simulink model "furuta_observer_loop"  (R2024b)
settings: Solver=ode45  StartTime=0.0  StopTime=4  MaxStep=1e-3  RelTol=1e-3
values from neighbouring files (symbols this model uses):
  L = place(A', C', p_obs)'    [furuta_observer.m]
  tap_amp = 1    [furuta_no_observer.m]    (also in furuta_observer.m)
  tap_len = 0.1    [furuta_no_observer.m]    (also in furuta_observer.m)
  tap_time = 2    [furuta_no_observer.m]    (also in furuta_observer.m)
  Vmax = 10    [furuta_no_observer.m]    (also in furuta_observer.m)
  x0 = [0; deg2rad(10); 0; 0]    [furuta_no_observer.m]    (also in furuta_observer.m)
  xhat0 = zeros(4,1)    [furuta_observer.m]
undefined symbols (not defined in the file or in its folder): A, B, C, K
settings Model: Creator=alekseiprakhiy  LastModifiedBy=alekseiprakhiy

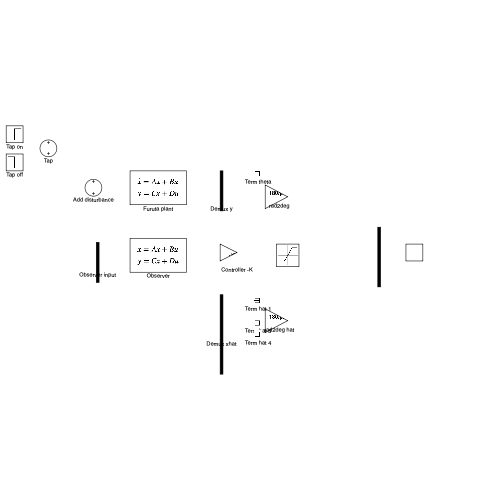
[thumbnail: Simulink's stored preview of the top-level diagram]
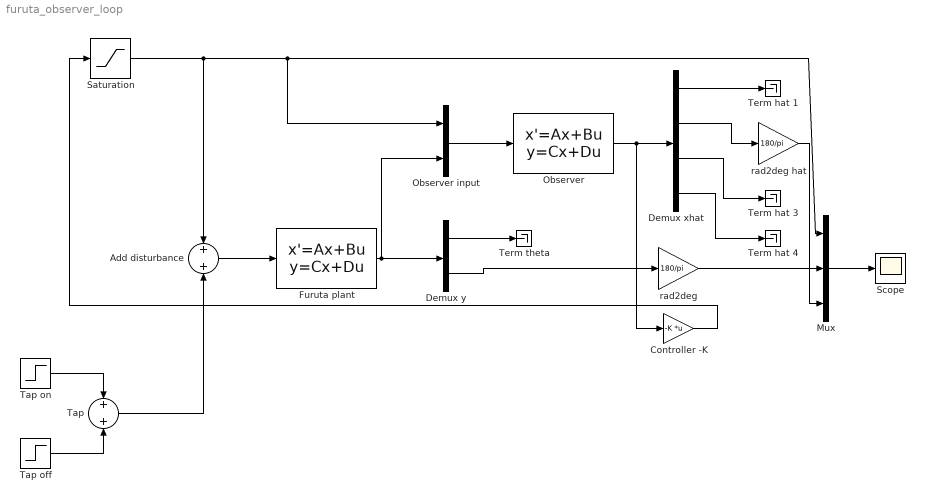
== system furuta_observer_loop ==
  Add disturbance : Sum
  Controller -K : Gain  Gain=-K  Multiplication=Matrix(K*u)
  Demux xhat : Demux
  Demux y : Demux  Outputs=2
  Furuta plant : StateSpace  A=A  B=B  C=C  D=zeros(2,1)  InitialCondition=x0
  Mux : Mux  Inputs=3
  Observer : StateSpace  A=A - L*C  B=[B L]  C=eye(4)  D=zeros(4,3)  InitialCondition=xhat0
  Observer input : Mux  Inputs=2
  Saturation : Saturate  UpperLimit=Vmax  LowerLimit=-Vmax
  Scope : Scope
  Tap : Sum
  Tap off : Step  Time=tap_time + tap_len  After=-tap_amp  SampleTime=0
  Tap on : Step  Time=tap_time  After=tap_amp  SampleTime=0
  Term hat 1 : Terminator
  Term hat 3 : Terminator
  Term hat 4 : Terminator
  Term theta : Terminator
  rad2deg : Gain  Gain=180/pi
  rad2deg hat : Gain  Gain=180/pi
  wires:
  rad2deg hat/1 -> Mux/3
  rad2deg/1 -> Mux/2
  Demux xhat/4 -> Term hat 4/1
  Demux xhat/2 -> rad2deg hat/1
  Furuta plant/1 -> Demux y/1, Observer input/2
  Mux/1 -> Scope/1
  Tap off/1 -> Tap/2
  Demux xhat/1 -> Term hat 1/1
  Add disturbance/1 -> Furuta plant/1
  Saturation/1 -> Observer input/1, Mux/1, Add disturbance/1
  Demux y/1 -> Term theta/1
  Tap/1 -> Add disturbance/2
  Demux xhat/3 -> Term hat 3/1
  Observer/1 -> Demux xhat/1, Controller -K/1
  Demux y/2 -> rad2deg/1
  Observer input/1 -> Observer/1
  Controller -K/1 -> Saturation/1
  Tap on/1 -> Tap/1
